simulink model "ss3_dryer_loads"  (R2024b)
settings: Solver=ode45  StartTime=0.0  StopTime=28800  MaxStep=1  MinStep=0.001  RelTol=1e-3
undefined symbols (not defined in the file): DRY
settings Model: Creator=user  LastModifiedBy=user

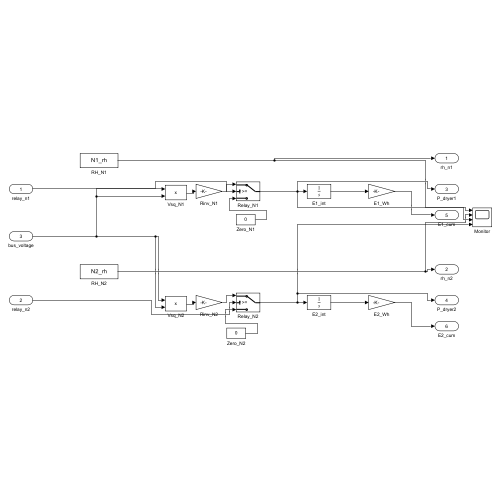
[thumbnail: Simulink's stored preview of the top-level diagram]
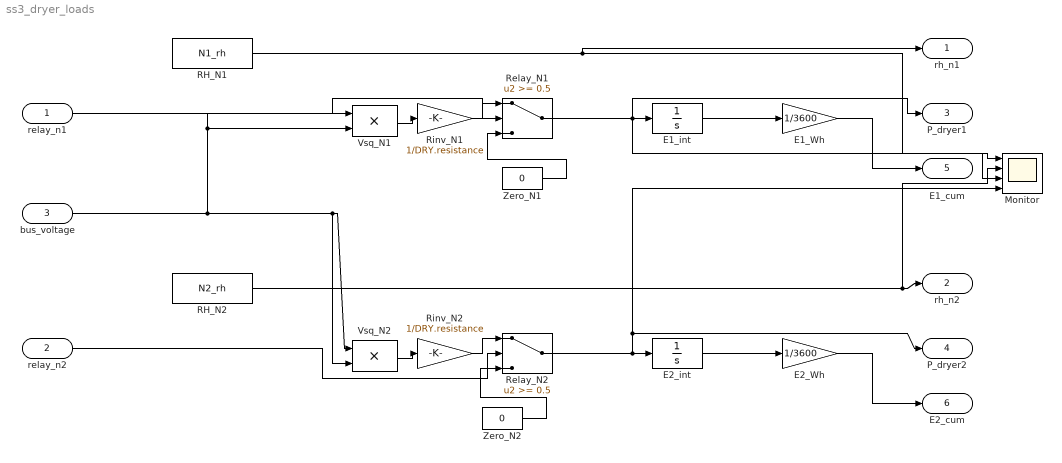
== system ss3_dryer_loads ==
  relay_n1 : Inport
  relay_n2 : Inport  Port=2
  bus_voltage : Inport  Port=3
  E1_Wh : Gain  Gain=1/3600
  E1_int : Integrator
  E2_Wh : Gain  Gain=1/3600
  E2_int : Integrator
  Monitor : Scope  NumInputPorts=4
  RH_N1 : FromWorkspace  VariableName=N1_rh
  RH_N2 : FromWorkspace  VariableName=N2_rh
  Relay_N1 : Switch  Threshold=0.5  SaturateOnIntegerOverflow=off  InputSameDT=off
  Relay_N2 : Switch  Threshold=0.5  SaturateOnIntegerOverflow=off  InputSameDT=off
  Rinv_N1 : Gain  Gain=1/DRY.resistance
  Rinv_N2 : Gain  Gain=1/DRY.resistance
  Vsq_N1 : Product  Inputs=**
  Vsq_N2 : Product  Inputs=**
  Zero_N1 : Constant  Value=0
  Zero_N2 : Constant  Value=0
  rh_n1 : Outport
  rh_n2 : Outport  Port=2
  P_dryer1 : Outport  Port=3
  P_dryer2 : Outport  Port=4
  E1_cum : Outport  Port=5
  E2_cum : Outport  Port=6
  wires:
  bus_voltage/1 -> Vsq_N2/1, Vsq_N2/2, Vsq_N1/1, Vsq_N1/2
  Vsq_N1/1 -> Rinv_N1/1
  Vsq_N2/1 -> Rinv_N2/1
  Rinv_N1/1 -> Relay_N1/1
  Rinv_N2/1 -> Relay_N2/1
  relay_n1/1 -> Relay_N1/2
  relay_n2/1 -> Relay_N2/2
  Zero_N1/1 -> Relay_N1/3
  Zero_N2/1 -> Relay_N2/3
  Relay_N1/1 -> E1_int/1, P_dryer1/1, Monitor/3
  Relay_N2/1 -> P_dryer2/1, Monitor/4, E2_int/1
  E1_int/1 -> E1_Wh/1
  E2_int/1 -> E2_Wh/1
  RH_N1/1 -> rh_n1/1, Monitor/1
  RH_N2/1 -> rh_n2/1, Monitor/2
  E1_Wh/1 -> E1_cum/1
  E2_Wh/1 -> E2_cum/1
